simulink model "Quad_UAV_Dynamics_R2024a"  (R2024a)
settings: Solver=VariableStepAuto  StartTime=0.0  StopTime=inf  RelTol=1e-3
PreLoadFcn:
  | InitVars;
values from neighbouring files (symbols this model uses):
  dragCoeffMov = diag([0.1, 0.1, 0.2])    [InitVars.m]
  g = 9.80665    [InitVars.m]
  m_to_mm = 1000    [InitVars.m]
  mass = 1.0    (= 1)    [InitVars.m]
  ms2_to_mg = 1000 / g    (= 101.971621298)    [InitVars.m]
  ms_to_cms = 100    [InitVars.m]
  ref_height = 488.0    (= 488)    [InitVars.m]
  ref_lat = 47.397742    [InitVars.m]
  ref_lon = 8.545594    [InitVars.m]
  rotorDir = [-1; -1; 1; 1]    [InitVars.m]
  rotorPositions = [ armLength*cos(pi/4), -armLength*sin(pi/4), 0 ... (first row only)    [InitVars.m]
  rotorThrustMax = 5.0    (= 5)    [InitVars.m]
  rotorTimeConst = 0.05    [InitVars.m]
  rotorTorqueMax = 0.05    [InitVars.m]
  SampleTime = 0.005    [InitVars.m]    (also in px4HostTarget_TCPIP_Read.m = -1)
  windVel = [0; 0; 0]    [InitVars.m]
undefined symbols (not defined in the file or in its folder): contact, control, fractalcoef, Payload, uav
libraries: uavmavlinklib x5, simulink x2, sharedtransform x2, aerolibatmos2 x1, sensorgpslib x1, robotcorelib x1, mspsensorlib x1, shared6dof x1, uavutilslib x1
(part 1 of 2)
settings Model: LastModifiedBy=LOQ
settings OptimizationCC: BlockReduction=off  BooleanDataType=off
settings DebuggingCC: SaveWithParameterizedLinksMsg=none  UnderspecifiedInitializationDetection=Classic  MergeDetectMultiDrivingBlocksExec=none  SignalResolutionControl=TryResolveAllWithWarning
settings HardwareCC: TargetUnknown=on
settings ModelReferenceCC: PropagateSignalLabelsOutOfModel=off

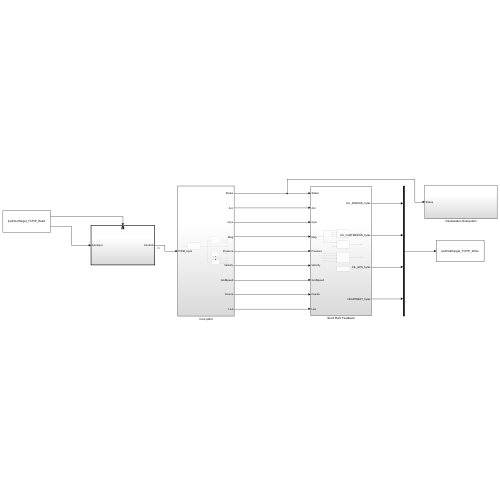
[thumbnail: Simulink's stored preview of the top-level diagram]
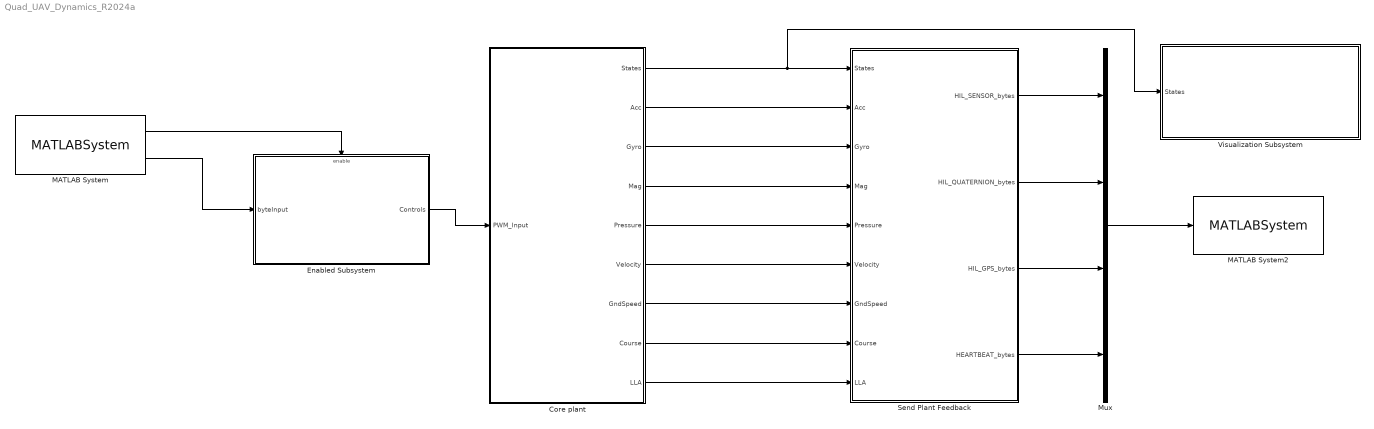
== system Quad_UAV_Dynamics_R2024a ==
  Core plant : Subsystem
  Enabled Subsystem : Subsystem  TreatAsAtomicUnit=on
  MATLAB System : MATLABSystem  System=px4HostTarget_TCPIP_Read  Length=50  SampleTime=SampleTime
      mask Type: px4HostTarget_TCPIP_Read
      mask Display:
      | color('white');
      | plot([100,100,100,100]*1,[100,100,100,100]*1);
      | plot([100,100,100,100]*0,[100,100,100,100]*0);
      | color('black');
      | text(50,50,'TCP Read','horizontalAlignment','center');
      | text(50,12,sprintf('Port: %d',4560) ,'horizontalAlignment', 'center');
      | port_label('output',1,'Status');
      | port_label('output',2,'Data');
  MATLAB System2 : MATLABSystem  System=px4HostTarget_TCPIP_Write
      mask Type: px4HostTarget_TCPIP_Write
      mask Display:
      | color('white');
      | plot([100,100,100,100]*1,[100,100,100,100]*1);
      | plot([100,100,100,100]*0,[100,100,100,100]*0);
      | color('black');
      | sppkgroot = strrep(codertarget.pixhawk.internal.getSpPkgRootDir(),'\','/');
      | image(fullfile(sppkgroot,'resources','TCP.jpg'),'center')
      | color('black');
      | text(50,12,sprintf('Port: %d',4560) ,'horizontalAlignment', 'center');
  Mux : Mux
  Send Plant Feedback : Subsystem
  Visualization Subsystem : Subsystem
  wires:
  MATLAB System/1 -> Enabled Subsystem/Enable
  MATLAB System/2 -> Enabled Subsystem/1(byteInput)
  Enabled Subsystem/1(Controls) -> Core plant/1(PWM_Input)
  Core plant/2(Acc) -> Send Plant Feedback/2(Acc)
  Core plant/3(Gyro) -> Send Plant Feedback/3(Gyro)
  Core plant/4(Mag) -> Send Plant Feedback/4(Mag)
  Core plant/1(States) -> Visualization Subsystem/1(States), Send Plant Feedback/1(States)
  Core plant/5(Pressure) -> Send Plant Feedback/5(Pressure)
  Core plant/6(Velocity) -> Send Plant Feedback/6(Velocity)
  Core plant/7(GndSpeed) -> Send Plant Feedback/7(GndSpeed)
  Core plant/8(Course) -> Send Plant Feedback/8(Course)
  Core plant/9(LLA) -> Send Plant Feedback/9(LLA)
  Send Plant Feedback/1(HIL_SENSOR_bytes) -> Mux/1
  Send Plant Feedback/2(HIL_QUATERNION_bytes) -> Mux/2
  Send Plant Feedback/3(HIL_GPS_bytes) -> Mux/3
  Send Plant Feedback/4(HEARTBEAT_bytes) -> Mux/4
  Mux/1 -> MATLAB System2/1

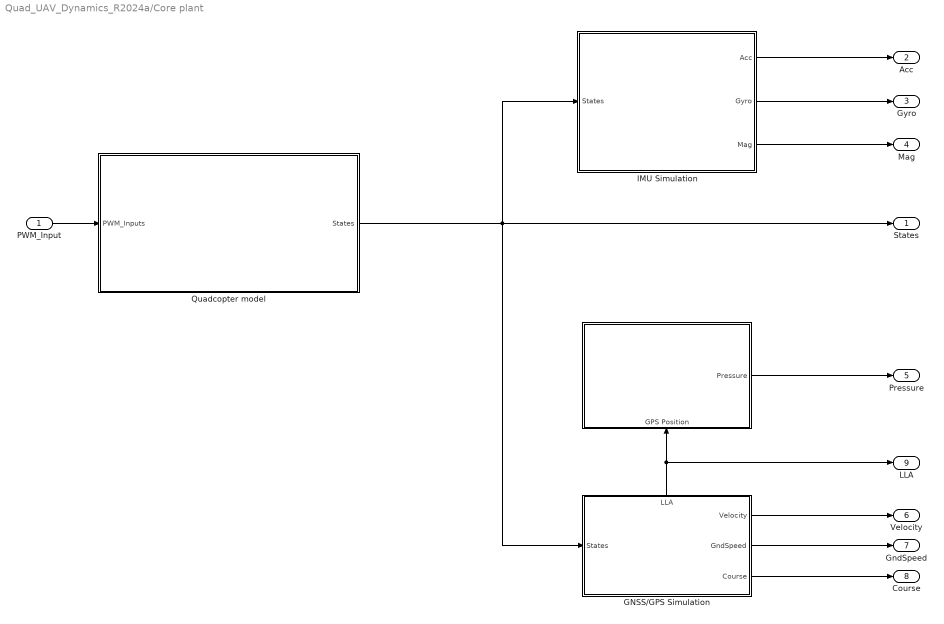
== system Quad_UAV_Dynamics_R2024a/Core plant ==
  PWM_Input : Inport  OutDataTypeStr=double  PortDimensions=[1 4]
  " " : Subsystem
      settings: PortSchema="{\"entries\":[{\"content\":{\"sides\":[{\"content\":{\"connectorIds\":[]},\"type\":\"ConnectorPlacement.EquallySpacedRectSide\",\"uuid\":\"7ecc8b21-8f8f-4144-826a-6b68e30dbf7d\"},{\"content\":{\"connectorIds\":[\"Out1\"],\"side\":\"RIGHT\"},\"type\":\"ConnectorPlacement.EquallySpacedRectSide\",\"uuid\":\"81a1dd55-8330-4386-9921-36c0eb60d526\"},{\"content\":{\"connectorIds\":[],\"side\":\"TOP\"},\"type\":\"ConnectorPlacement.EquallySpacedRectSide\",\"uuid\":\"b99caff5-b40d-407d-b30e-35210c1aee1d\"},{\"content\":{\"connectorIds\":[\"In1\"],\"side\":\"BOTTOM\"},\"type\":\"ConnectorPlacement.EquallySpacedRectSide\",\"uuid\":\"18bfda3d-4fab-4e61-9ebc-e384e51de306\"}]},\"type\":\"ConnectorPlacement.EquallySpacedConnector\",\"uuid\":\"17ab4e96-b761-4c62-a0bb-ab626dac3eaa\"}],\"packageUris\":[\"http://schema.mathworks.com/mf0/Connector/R2020b\"],\"version\":\"1.0\"}"
  GNSS/GPS Simulation : Subsystem
      settings: PortSchema="{\"entries\":[{\"content\":{\"sides\":[{\"content\":{\"connectorIds\":[\"In1\"]},\"type\":\"ConnectorPlacement.EquallySpacedRectSide\",\"uuid\":\"4934e8ff-5d4b-4e11-968d-c23bd62383a0\"},{\"content\":{\"connectorIds\":[\"Out1\",\"Out2\",\"Out3\"],\"side\":\"RIGHT\"},\"type\":\"ConnectorPlacement.EquallySpacedRectSide\",\"uuid\":\"9ec8bc0a-2d3c-4dca-835c-010ac29b6ebc\"},{\"content\":{\"connectorIds\":[\"Out4\"],\"side\":\"TOP\"},\"type\":\"ConnectorPlacement.EquallySpacedRectSide\",\"uuid\":\"04f09eb4-1bd9-450e-b951-47054bdd92ad\"}]},\"type\":\"ConnectorPlacement.EquallySpacedConnector\",\"uuid\":\"9a5920cf-a58d-4c98-839b-fbac94edbe7e\"}],\"packageUris\":[\"http://schema.mathworks.com/mf0/Connector/R2020b\"],\"version\":\"1.0\"}"
  IMU Simulation : Subsystem
      settings: PortSchema="{\"entries\":[{\"content\":{\"sides\":[{\"content\":{},\"type\":\"ConnectorPlacement.EquallySpacedRectSide\",\"uuid\":\"0f5c2282-ad4e-4c27-a92f-532c88dd9b34\"},{\"content\":{\"side\":\"RIGHT\"},\"type\":\"ConnectorPlacement.EquallySpacedRectSide\",\"uuid\":\"b1a389a9-bd19-4f0a-ab56-19663216dbdf\"},{\"content\":{\"connectorIds\":[\"In1\"],\"side\":\"TOP\"},\"type\":\"ConnectorPlacement.EquallySpacedRectSide\",\"uuid\":\"61bb26dd-3b4e-45d7-8996-b1e12f9a0a9d\"},{\"content\":{\"connectorIds\":[\"Out1\",\"Out2\",\"Out3\"],\"side\":\"BOTTOM\"},\"type\":\"ConnectorPlacement.EquallySpacedRectSide\",\"uuid\":\"ba157af1-2ca4-4452-bdd7-6e3dad9cb5e7\"},{\"content\":{\"side\":\"HIDDEN\"},\"type\":\"ConnectorPlacement.EquallySpacedRectSide\",\"uuid\":\"fff182b3-fe96-4082-825e-95746cd3e6b2\"}]},\"type\":\"ConnectorPlacement.EquallySpacedConnector\",\"uuid\":\"8a88afc7-c2a2-4beb-8758-d3390628bed4\"}],\"packageUris\":[\"http://schema.mathworks.com/mf0/Connector/R2020b\"],\"version\":\"1.0\"}"
  Quadcopter model : Subsystem
  States : Outport
  Acc : Outport  Port=2
  Gyro : Outport  Port=3
  Mag : Outport  Port=4
  Pressure : Outport  Port=5
  Velocity : Outport  Port=6
  GndSpeed : Outport  Port=7
  Course : Outport  Port=8
  LLA : Outport  Port=9
  wires:
  IMU Simulation/3(Acc) -> Acc/1
  PWM_Input/1 -> Quadcopter model/1(PWM_Inputs)
  Quadcopter model/1(States) -> GNSS/GPS Simulation/1(States), States/1, IMU Simulation/1(States)
  IMU Simulation/2(Gyro) -> Gyro/1
  IMU Simulation/1(Mag) -> Mag/1
  GNSS/GPS Simulation/4(LLA) -> LLA/1, " "/1(GPS Position)
  " "/1(Pressure) -> Pressure/1
  GNSS/GPS Simulation/1(Velocity) -> Velocity/1
  GNSS/GPS Simulation/2(GndSpeed) -> GndSpeed/1
  GNSS/GPS Simulation/3(Course) -> Course/1

== system Quad_UAV_Dynamics_R2024a/Enabled Subsystem ==
  byteInput : Inport
  Enable : EnablePort
  Bus Selector : BusSelector  OutputSignals=Payload.controls
  Data Type Conversion : DataTypeConversion  OutDataTypeStr=double  SaturateOnIntegerOverflow=off  RndMeth=Floor
  Display : Display
  MAVLink Deserializer : uavmavlinklib/MAVLink Deserializer  dialectSource=Select from standard MAVLink dialects  dialect=common.xml  dialectCustom=common.xml  version=2  messageType=HIL_ACTUATOR_CONTROLS  inputDataLength=off  SystemIDFilter=off  systemID=1  ComponentIDFilter=off  componentID=1  queueMsg=off  queueMsgSize=50  dropNum=off
  Selector1 : Selector  InputPortWidth=16  IndexOptions=Index vector (dialog)  Indices=[1:4]  OutputSizes=1
  Controls : Outport
  wires:
  byteInput/1 -> MAVLink Deserializer/1
  MAVLink Deserializer/2 -> Bus Selector/1
  Bus Selector/1 -> Data Type Conversion/1  "<controls>"
  MAVLink Deserializer/1 -> Display/1  "status"
  Data Type Conversion/1 -> Selector1/1
  Selector1/1 -> Controls/1

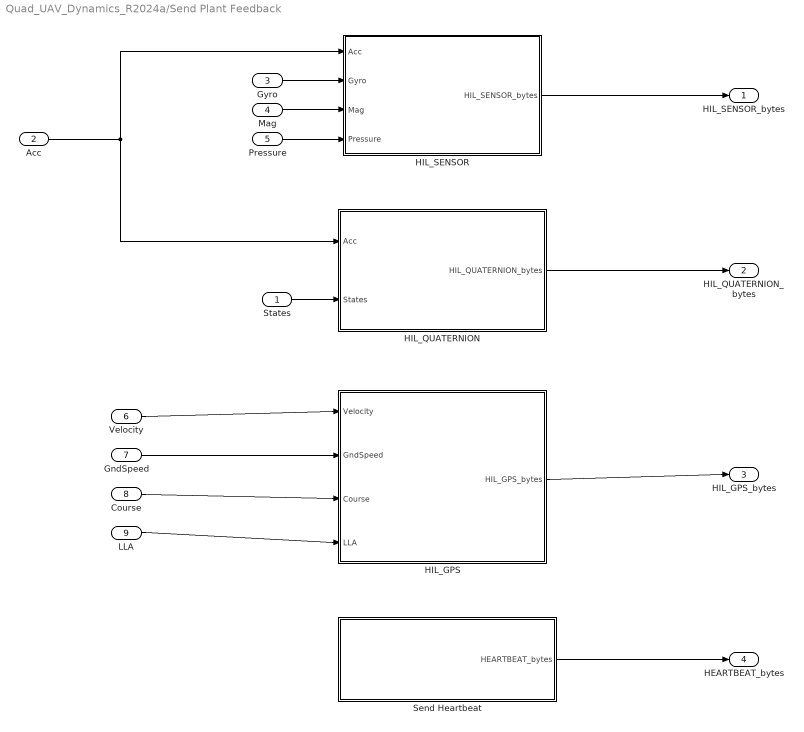
== system Quad_UAV_Dynamics_R2024a/Send Plant Feedback ==
  States : Inport
  Acc : Inport  Port=2
  Gyro : Inport  Port=3
  Mag : Inport  Port=4
  Pressure : Inport  Port=5
  Velocity : Inport  Port=6
  GndSpeed : Inport  Port=7
  Course : Inport  Port=8
  LLA : Inport  Port=9
  HIL_GPS : Subsystem
  HIL_QUATERNION : Subsystem
  HIL_SENSOR : Subsystem
  Send Heartbeat : Subsystem
  HIL_SENSOR_bytes : Outport
  HIL_QUATERNION_bytes : Outport  Port=2
  HIL_GPS_bytes : Outport  Port=3
  HEARTBEAT_bytes : Outport  Port=4
  wires:
  Pressure/1 -> HIL_SENSOR/4(Pressure)
  Acc/1 -> HIL_SENSOR/1(Acc), HIL_QUATERNION/1(Acc)
  States/1 -> HIL_QUATERNION/2(States)
  Mag/1 -> HIL_SENSOR/3(Mag)
  GndSpeed/1 -> HIL_GPS/2(GndSpeed)
  Gyro/1 -> HIL_SENSOR/2(Gyro)
  HIL_SENSOR/1(HIL_SENSOR_bytes) -> HIL_SENSOR_bytes/1
  HIL_QUATERNION/1(HIL_QUATERNION_bytes) -> HIL_QUATERNION_bytes/1
  Course/1 -> HIL_GPS/3(Course)
  Velocity/1 -> HIL_GPS/1(Velocity)
  LLA/1 -> HIL_GPS/4(LLA)
  HIL_GPS/1(HIL_GPS_bytes) -> HIL_GPS_bytes/1
  Send Heartbeat/1(HEARTBEAT_bytes) -> HEARTBEAT_bytes/1

== system Quad_UAV_Dynamics_R2024a/Visualization Subsystem ==
  States : Inport
  Bus Selector : BusSelector  OutputSignals=X,Y,Z  OutputAsBus=on
  Bus Selector1 : BusSelector  OutputSignals=yaw,pitch,roll  OutputAsBus=on
  Rotation Angles to Quaternions : sharedtransform/Rotation Angles to Quaternions  rotationOrder=ZYX  aMode=aMode
  UAV Animation : uavutilslib/UAV Animation  UAVType=Multirotor  UAVSize=1  InertialZDirection=Down  SampleTime=-1
  wires:
  Bus Selector/1 -> UAV Animation/1
  Rotation Angles to Quaternions/1 -> UAV Animation/2
  Bus Selector1/1 -> Rotation Angles to Quaternions/1
  States/1 -> Bus Selector1/1, Bus Selector/1

== system Quad_UAV_Dynamics_R2024a/Core plant/  ==
  GPS Position : Inport
  Extract Altitude : Selector  InputPortWidth=3  IndexOptions=Index vector (dialog)  Indices=[3]  OutputSizes=1
  Gain1 : Gain  Gain=1/m_to_mm
  Gain2 : Gain  Gain=m_to_mm
  Lapse Rate Model : aerolibatmos2/ISA Atmosphere Model  useExtended=off  action=Warning  custom=on  viscosityOut=off  g=9.80665  gamma=1.4  R=287.0531  L=0.0065  h_trop=11000  h_strat=20000  rho0=1.225  P0=101325  T0=288.15  h0=0  S=110.4  Tref=273.15  muref=1.716e-5
  Random Number1 : RandomNumber  Variance=10000  Seed=10  SampleTime=SampleTime
  Sum1 : Sum  Inputs=|++
  Terminator : Terminator
  Terminator1 : Terminator
  Terminator2 : Terminator
  Pressure : Outport
  wires:
  Lapse Rate Model/2 -> Terminator1/1
  Lapse Rate Model/4 -> Terminator2/1
  Lapse Rate Model/1 -> Terminator/1
  Lapse Rate Model/3 -> Pressure/1
  Sum1/1 -> Gain1/1
  Gain2/1 -> Sum1/1
  Extract Altitude/1 -> Gain2/1
  Gain1/1 -> Lapse Rate Model/1
  GPS Position/1 -> Extract Altitude/1
  Random Number1/1 -> Sum1/2  "Pressure_noise"

== system Quad_UAV_Dynamics_R2024a/Core plant/GNSS//GPS Simulation ==
  States : Inport
  Bus Selector : BusSelector  OutputSignals=dx,dy,dz  OutputAsBus=on
  Bus Selector1 : BusSelector  OutputSignals=X,Y,Z  OutputAsBus=on
  GPS : sensorgpslib/GPS  DispRefFrame=NED  PositionInputFormat=Local  ReferenceLocation=[ref_lat ref_lon ref_height]  HorizontalPositionAccuracy=0.01  VerticalPositionAccuracy=0.01  VelocityAccuracy=0.01  DecayFactor=0.99  SeedDouble=67  SimulateUsing=Interpreted execution
  Reshape1 : Reshape  OutputDimensionality=Row vector (2-D)
  Reshape3 : Reshape  OutputDimensionality=Row vector (2-D)
  Velocity : Outport
  GndSpeed : Outport  Port=2
  Course : Outport  Port=3
  LLA : Outport  Port=4
  wires:
  Reshape3/1 -> GPS/1
  GPS/1 -> LLA/1  "lla"
  Bus Selector1/1 -> Reshape3/1
  Bus Selector/1 -> Reshape1/1
  Reshape1/1 -> GPS/2
  GPS/2 -> Velocity/1
  States/1 -> Bus Selector/1, Bus Selector1/1
  GPS/3 -> GndSpeed/1
  GPS/4 -> Course/1

== system Quad_UAV_Dynamics_R2024a/Core plant/IMU Simulation ==
  States : Inport
  IMU Subsystem : Subsystem
  Mag : Outport
  Gyro : Outport  Port=2
  Acc : Outport  Port=3
  wires:
  States/1 -> IMU Subsystem/1(States)
  IMU Subsystem/1(Acc) -> Acc/1
  IMU Subsystem/2(Gyro) -> Gyro/1
  IMU Subsystem/3(Mag) -> Mag/1

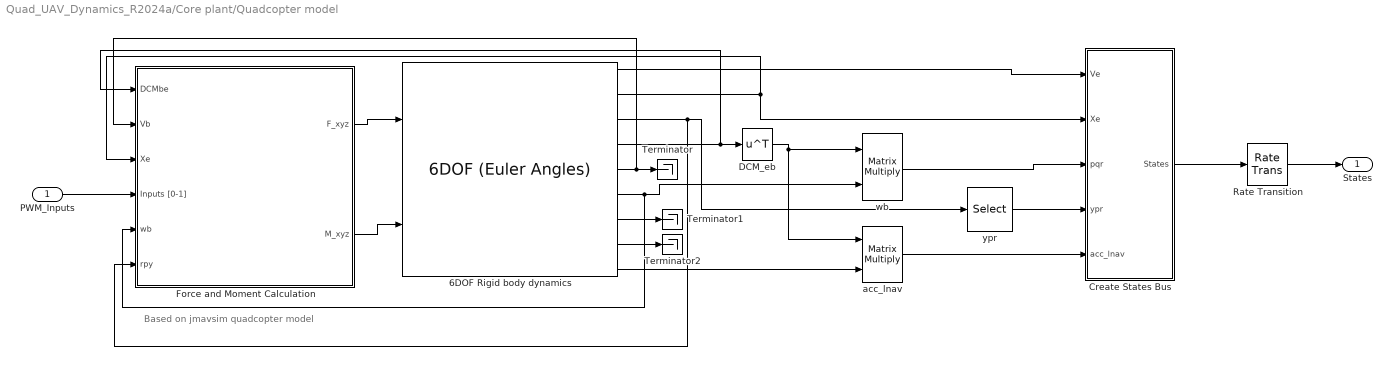
== system Quad_UAV_Dynamics_R2024a/Core plant/Quadcopter model ==
  note: Based on jmavsim quadcopter model
  PWM_Inputs : Inport
  "6DOF Rigid body dynamics " : shared6dof/6DOF (Euler Angles)  units=Metric (MKS)  mtype=Fixed  rep=Euler Angles  xme_0=init.posNED  Vm_0=init.vb  eul_0=init.euler  pm_0=init.angRates  mass_0=mass  mass_e=0.5  mass_f=2.0  inertia=inertia  inertia_e=eye(3)  inertia_f=2*eye(3)  k_quat=Vehicle.SixDOF.quatGain  vre_flag=on  abi_flag=on  aMode=aMode  xme_statename=''  Vm_statename=''  eul_statename=''  quat_statename=''  pm_statename=''  mass_statename=''
  Create States Bus : Subsystem
  DCM_eb : Math  Operator=transpose
  Force and Moment Calculation : Subsystem
  Rate Transition : RateTransition  OutPortSampleTime=SampleTime
  Terminator : Terminator
  Terminator1 : Terminator
  Terminator2 : Terminator
  acc_lnav : Product  Multiplication=Matrix(*)
  wb : Product  Multiplication=Matrix(*)
  ypr : Selector  InputPortWidth=3  IndexOptions=Index vector (dialog)  Indices=[3 2 1]  OutputSizes=1
  States : Outport
  wires:
  "6DOF Rigid body dynamics "/3 -> Force and Moment Calculation/6(rpy), ypr/1
  Force and Moment Calculation/1(F_xyz) -> "6DOF Rigid body dynamics "/1
  Force and Moment Calculation/2(M_xyz) -> "6DOF Rigid body dynamics "/2
  Rate Transition/1 -> States/1
  "6DOF Rigid body dynamics "/1 -> Create States Bus/1(Ve)
  PWM_Inputs/1 -> Force and Moment Calculation/4(Inputs [0-1])
  ypr/1 -> Create States Bus/4(ypr)
  Create States Bus/1(States) -> Rate Transition/1
  "6DOF Rigid body dynamics "/4 -> DCM_eb/1, Force and Moment Calculation/1(DCMbe)
  "6DOF Rigid body dynamics "/2 -> Force and Moment Calculation/3(Xe), Create States Bus/2(Xe)
  "6DOF Rigid body dynamics "/6 -> Force and Moment Calculation/5(wb), wb/2
  wb/1 -> Create States Bus/3(pqr)
  DCM_eb/1 -> acc_lnav/1, wb/1
  "6DOF Rigid body dynamics "/9 -> acc_lnav/2
  acc_lnav/1 -> Create States Bus/5(acc_lnav)
  "6DOF Rigid body dynamics "/5 -> Force and Moment Calculation/2(Vb), Terminator/1
  "6DOF Rigid body dynamics "/7 -> Terminator1/1
  "6DOF Rigid body dynamics "/8 -> Terminator2/1

== system Quad_UAV_Dynamics_R2024a/Send Plant Feedback/HIL_GPS ==
  Velocity : Inport
  GndSpeed : Inport  Port=2
  Course : Inport  Port=3
  LLA : Inport  Port=4
  HIL_GPS Subsystem : Subsystem
  MAVLink Serializer3 : uavmavlinklib/MAVLink Serializer  dialectSource=Select from standard MAVLink dialects  dialect=common.xml  dialectCustom=common.xml  version=2  messageType=HIL_GPS
  Terminator3 : Terminator
  HIL_GPS_bytes : Outport
  wires:
  Course/1 -> HIL_GPS Subsystem/4(Course)
  Velocity/1 -> HIL_GPS Subsystem/2(Velocity)
  MAVLink Serializer3/2 -> Terminator3/1
  HIL_GPS Subsystem/1(Out1) -> MAVLink Serializer3/1
  MAVLink Serializer3/1 -> HIL_GPS_bytes/1
  LLA/1 -> HIL_GPS Subsystem/1(LLA)
  GndSpeed/1 -> HIL_GPS Subsystem/3(GndSpeed)

== system Quad_UAV_Dynamics_R2024a/Send Plant Feedback/HIL_QUATERNION ==
  Acc : Inport
  States : Inport  Port=2
  GPS Subsystem : Subsystem
      settings: PortSchema="{\"entries\":[{\"content\":{\"sides\":[{\"content\":{\"connectorIds\":[\"In1\"]},\"type\":\"ConnectorPlacement.EquallySpacedRectSide\",\"uuid\":\"bd7d303d-974a-4dd9-8d27-04cf87176bd7\"},{\"content\":{\"connectorIds\":[\"Out1\"],\"side\":\"RIGHT\"},\"type\":\"ConnectorPlacement.EquallySpacedRectSide\",\"uuid\":\"9b60b4cf-af27-4ca7-86b7-e75d27668f15\"},{\"content\":{\"connectorIds\":[\"In2\"],\"side\":\"TOP\"},\"type\":\"ConnectorPlacement.EquallySpacedRectSide\",\"uuid\":\"cd4d20a6-3033-4c65-942d-f02a7fa933e8\"},{\"content\":{\"side\":\"BOTTOM\"},\"type\":\"ConnectorPlacement.EquallySpacedRectSide\",\"uuid\":\"d837ff15-3ee7-4ba9-aab0-0378a7633b3a\"},{\"content\":{\"side\":\"HIDDEN\"},\"type\":\"ConnectorPlacement.EquallySpacedRectSide\",\"uuid\":\"eefe2c49-f98f-4c11-8e75-b071b558b610\"}]},\"type\":\"ConnectorPlacement.EquallySpacedConnector\",\"uuid\":\"bd9fca06-cb18-49af-bec9-4d4823ab7b04\"}],\"packageUris\":[\"http://schema.mathworks.com/mf0/Connector/R2020b\"],\"version\":\"1.0\"}"
  MAVLink Serializer2 : uavmavlinklib/MAVLink Serializer  dialectSource=Select from standard MAVLink dialects  dialect=common.xml  dialectCustom=common.xml  version=2  messageType=HIL_STATE_QUATERNION
  Terminator2 : Terminator
  HIL_QUATERNION_bytes : Outport
  wires:
  States/1 -> GPS Subsystem/1(States)
  MAVLink Serializer2/2 -> Terminator2/1
  GPS Subsystem/1(HIL Quaternion) -> MAVLink Serializer2/1
  MAVLink Serializer2/1 -> HIL_QUATERNION_bytes/1
  Acc/1 -> GPS Subsystem/2(Acc)

== system Quad_UAV_Dynamics_R2024a/Send Plant Feedback/HIL_SENSOR ==
  Acc : Inport
  Gyro : Inport  Port=2
  Mag : Inport  Port=3
  Pressure : Inport  Port=4
  Hil Sensor Creation subsystem : Subsystem
  MAVLink Serializer1 : uavmavlinklib/MAVLink Serializer  dialectSource=Select from standard MAVLink dialects  dialect=common.xml  dialectCustom=common.xml  version=2  messageType=HIL_SENSOR
  Terminator1 : Terminator
  HIL_SENSOR_bytes : Outport
  wires:
  MAVLink Serializer1/2 -> Terminator1/1
  Hil Sensor Creation subsystem/1(HIL Sensor) -> MAVLink Serializer1/1
  Acc/1 -> Hil Sensor Creation subsystem/1(Acc)
  MAVLink Serializer1/1 -> HIL_SENSOR_bytes/1
  Gyro/1 -> Hil Sensor Creation subsystem/2(Gyro)
  Mag/1 -> Hil Sensor Creation subsystem/3(Mag)
  Pressure/1 -> Hil Sensor Creation subsystem/4(Pressure)

== system Quad_UAV_Dynamics_R2024a/Send Plant Feedback/Send Heartbeat ==
  Bus Assignment : BusAssignment  AssignedSignals=Payload.autopilot,Payload.type
  Constant : Constant  SampleTime=SampleTime
  Constant1 : Constant  Value=12  SampleTime=SampleTime
  Data Type Conversion : DataTypeConversion  OutDataTypeStr=uint8  SaturateOnIntegerOverflow=off  RndMeth=Floor
  Data Type Conversion1 : DataTypeConversion  OutDataTypeStr=uint8  SaturateOnIntegerOverflow=off  RndMeth=Floor
  MAVLink Blank Message : Subsystem  InitFcn=uav.sluav.internal.mavlink.util.errorIfBlocksConflict(bdroot(gcb))  mask(MAVLink Blank Message){dialectSource=Select from standard MAVLink dialects, dialect=common.xml, dialectCustom=common.xml, version=2, messageType=HEARTBEAT, SystemID=2, ComponentID=51, SampleTime=SampleTime}
      mask prompts: dialectSource "uav:robotsluav:mavlink:DialectSourcePrompt"; dialect "uav:robotsluav:mavlink:DialectPrompt"; dialectCustom "uav:robotsluav:mavlink:DialectPromptCustom"; version "uav:robotsluav:mavlink:VersionPrompt"; messageType "uav:robotsluav:mavlink:MessageTypePrompt"; SystemID "uav:robotsluav:mavlink:EnterSystemIDPrompt"; ComponentID "uav:robotsluav:mavlink:EnterComponentIDPrompt"; SampleTime "Simulink:blkprm_prompts:AllSrcBlksSampleTime"
      mask help: uav:robotsluav:mavlink:BlankMessageDescription
      mask init:
      | uav.sluav.internal.mavlink.block.MessageBlockMask.dispatch('maskInitialize', gcb)
      settings: LibrarySourceBlock=uavmavlinklib/MAVLink Blank Message  ModelCloseFcn=uav.sluav.internal.mavlink.block.MessageBlockMask.dispatch('modelCloseFcn', gcb);
      mask Help: eval("helpview('uav','uavMAVLinkBlankMessage')");
      mask TypeOptions dialectSource: uav:robotsluav:mavlink:DialectSourceFromStandard | uav:robotsluav:mavlink:DialectSourceSpecifyOwn
      mask Callback dialectSource: uav.sluav.internal.mavlink.block.MessageBlockMask.dispatch('dialectSourceSelect', gcb);
      mask TypeOptions dialect: uav:robotsluav:mavlink:DialectCommon | uav:robotsluav:mavlink:DialectArdupilotmega | uav:robotsluav:mavlink:DialectASLUAV | uav:robotsluav:mavlink:DialectAutoquad | uav:robotsluav:mavlink:DialectIcarous | uav:robotsluav:mavlink:DialectMatrixpilot | uav:robotsluav:mavlink:DialectMinimal | uav:robotsluav:mavlink:DialectPaparazzi | uav:robotsluav:mavlink:DialectSlugs | uav:robotsluav:mavlink:DialectStandard | uav:robotsluav:mavlink:DialectUalberta | uav:robotsluav:mavlink:DialectUAvionix
      mask Callback dialect: uav.sluav.internal.mavlink.block.MessageBlockMask.dispatch('dialectEdit', gcb);
      mask Callback dialectCustom: uav.sluav.internal.mavlink.block.MessageBlockMask.dispatch('dialectEdit', gcb);
      mask TypeOptions version: 2 | 1
      mask Callback version: uav.sluav.internal.mavlink.block.MessageBlockMask.dispatch('versionEdit', gcb);
      mask Callback messageType: uav.sluav.internal.mavlink.block.MessageBlockMask.dispatch('messageTypeEdit', gcb);
      mask Callback SystemID: uav.sluav.internal.mavlink.block.MessageBlockMask.dispatch('updateSystemAndComponentID', gcb);
      mask Callback ComponentID: uav.sluav.internal.mavlink.block.MessageBlockMask.dispatch('updateSystemAndComponentID', gcb);
      mask TypeOptions SampleTime: MsgIDConstant/SampleTime
      mask DialogControl MainContainer Prompt: uav:robotsluav:mavlink:MainTabTitle
      mask DialogControl dialectSource Prompt: MAVLink dialect source:
      mask DialogControl dialect Prompt: MAVLink dialect:
      mask DialogControl dialectCustom Prompt: MAVLink dialect:
      mask DialogControl dialectBrowseButton Prompt: uav:robotsluav:mavlink:DialectBrowsePrompt
      mask DialogControl dialectBrowseButton Callback: uav.sluav.internal.mavlink.block.MessageBlockMask.dispatch('dialectBrowse', gcb);
      mask DialogControl version Prompt: MAVLink version:
      mask DialogControl messageType Prompt: MAVLink message type:
      mask DialogControl msgSelectButton Prompt: uav:robotsluav:mavlink:MessageSelectPrompt
      mask DialogControl msgSelectButton Callback: uav.sluav.internal.mavlink.block.MessageBlockMask.dispatch('messageTypeSelect', gcb, 'uav.sluav.internal.mavlink.dlg.MessageTypeSelector');
      mask DialogControl SystemID Prompt: System ID:
      mask DialogControl ComponentID Prompt: Component ID:
      mask DialogControl SampleTime Prompt: Sample time:
      mask Display:
      | color('black');
      | text(0.5, 0.10, 'HEARTBEAT', 'horizontalAlignment', 'center');
      | port_label('output', 1, 'Msg');
  MAVLink Serializer : uavmavlinklib/MAVLink Serializer  dialectSource=Select from standard MAVLink dialects  dialect=common.xml  dialectCustom=common.xml  version=2  messageType=HEARTBEAT
  Terminator4 : Terminator
  HEARTBEAT_bytes : Outport
  wires:
  Bus Assignment/1 -> MAVLink Serializer/1
  Constant/1 -> Data Type Conversion/1
  MAVLink Serializer/1 -> HEARTBEAT_bytes/1
  Data Type Conversion1/1 -> Bus Assignment/3
  Data Type Conversion/1 -> Bus Assignment/2
  MAVLink Serializer/2 -> Terminator4/1
  Constant1/1 -> Data Type Conversion1/1
  MAVLink Blank Message/1(Out1) -> Bus Assignment/1

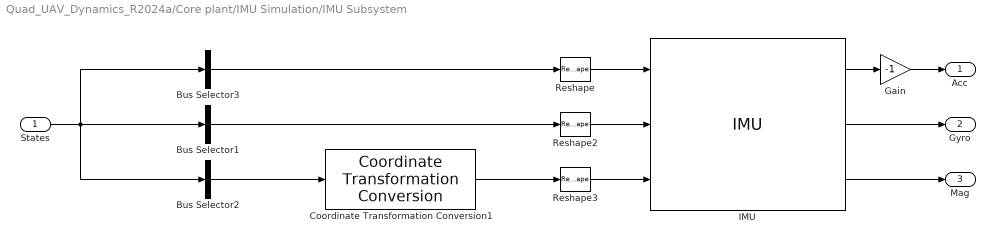
== system Quad_UAV_Dynamics_R2024a/Core plant/IMU Simulation/IMU Subsystem ==
  States : Inport
  Bus Selector1 : BusSelector  OutputSignals=p,q,r  OutputAsBus=on
  Bus Selector2 : BusSelector  OutputSignals=yaw,pitch,roll  OutputAsBus=on
  Bus Selector3 : BusSelector  OutputSignals=ddx,ddy,ddz  OutputAsBus=on
  Coordinate Transformation Conversion1 : robotcorelib/Coordinate Transformation Conversion  InputRepresentation=Euler Angles  InputEulerSequence=ZYX  ShowTrVecInputPort=on  OutputRepresentation=Quaternion  OutputEulerSequence=ZYX  ShowTrVecOutputPort=on  SimulateUsing=Interpreted execution
  Gain : Gain  Gain=-1
  IMU : mspsensorlib/IMU  DispRefFrame=NED  TemperaturePort=off  Temperature=25  MagneticFieldPort=off  MagneticFieldNED=[ 27.5550, -2.4169, -16.0849 ]  MagneticFieldENU=[ -2.4169, 27.5550, 16.0849 ]  SeedDouble=67  SimulateUsing=Interpreted execution  AccelParamsMeasurementRange=Inf  AccelParamsResolution=0  AccelParamsConstantBias=[ 0, 0, 0 ]  AccelParamsAxesMisalignment=[ 0, 0, 0 ]  AccelParamsNoiseDensity=[ 0, 0, 0 ]  AccelParamsBiasInstability=[ 0, 0, 0 ]  AccelParamsBiasInstabilityNumerator=fractalcoef().Numerator  AccelParamsBiasInstabilityDenominator=fractalcoef().Denominator  AccelParamsRandomWalk=[ 0, 0, 0 ]  AccelParamsNoiseType=double-sided  AccelParamsTemperatureBias=[ 0, 0, 0 ]  AccelParamsTemperatureScaleFactor=[ 0, 0, 0 ]  GyroParamsMeasurementRange=Inf  GyroParamsResolution=0  GyroParamsConstantBias=[ 0, 0, 0 ]  GyroParamsAxesMisalignment=[ 0, 0, 0 ]  GyroParamsAccelerationBias=[ 0, 0, 0 ]  GyroParamsNoiseDensity=[ 0, 0, 0 ]  GyroParamsBiasInstability=[ 0, 0, 0 ]  GyroParamsBiasInstabilityNumerator=fractalcoef().Numerator  GyroParamsBiasInstabilityDenominator=fractalcoef().Denominator  GyroParamsRandomWalk=[ 0, 0, 0 ]  GyroParamsNoiseType=double-sided  GyroParamsTemperatureBias=[ 0, 0, 0 ]  GyroParamsTemperatureScaleFactor=[ 0, 0, 0 ]  MagParamsMeasurementRange=Inf  MagParamsResolution=0  MagParamsConstantBias=[ 0, 0, 0 ]  MagParamsAxesMisalignment=[ 0, 0, 0 ]  MagParamsNoiseDensity=[ 0, 0, 0 ]  MagParamsBiasInstability=[ 0, 0, 0 ]  MagParamsBiasInstabilityNumerator=fractalcoef().Numerator  MagParamsBiasInstabilityDenominator=fractalcoef().Denominator  MagParamsRandomWalk=[ 0, 0, 0 ]  MagParamsNoiseType=double-sided  MagParamsTemperatureBias=[ 0, 0, 0 ]  MagParamsTemperatureScaleFactor=[ 0, 0, 0 ]
  Reshape : Reshape  OutputDimensionality=Row vector (2-D)
  Reshape2 : Reshape  OutputDimensionality=Row vector (2-D)
  Reshape3 : Reshape  OutputDimensionality=Row vector (2-D)
  Acc : Outport
  Gyro : Outport  Port=2
  Mag : Outport  Port=3
  wires:
  Bus Selector1/1 -> Reshape2/1
  IMU/1 -> Gain/1
  Bus Selector2/1 -> Coordinate Transformation Conversion1/1
  IMU/3 -> Mag/1
  Reshape2/1 -> IMU/2
  Bus Selector3/1 -> Reshape/1
  Coordinate Transformation Conversion1/1 -> Reshape3/1
  Reshape/1 -> IMU/1
  IMU/2 -> Gyro/1
  Reshape3/1 -> IMU/3
  States/1 -> Bus Selector3/1, Bus Selector2/1, Bus Selector1/1
  Gain/1 -> Acc/1

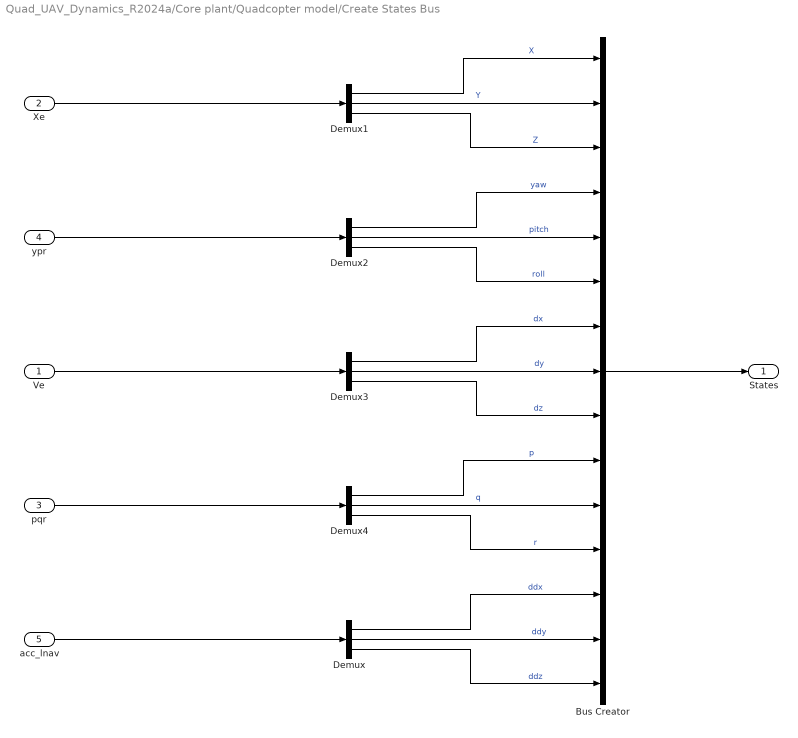
== system Quad_UAV_Dynamics_R2024a/Core plant/Quadcopter model/Create States Bus ==
  Ve : Inport
  Xe : Inport  Port=2
  pqr : Inport  Port=3
  ypr : Inport  Port=4
  acc_lnav : Inport  Port=5
  Bus Creator : BusCreator  Inputs=15
  Demux{,1..4} (5 alike) : Demux  Outputs=3
  States : Outport
  wires:
  Demux1/1 -> Bus Creator/1  "X"
  Demux1/2 -> Bus Creator/2  "Y"
  ypr/1 -> Demux2/1
  Demux2/2 -> Bus Creator/5  "pitch"
  Demux3/2 -> Bus Creator/8  "dy"
  Demux2/3 -> Bus Creator/6  "roll"
  pqr/1 -> Demux4/1
  Ve/1 -> Demux3/1
  Demux2/1 -> Bus Creator/4  "yaw"
  Demux1/3 -> Bus Creator/3  "Z"
  Demux3/1 -> Bus Creator/7  "dx"
  Demux4/2 -> Bus Creator/11  "q"
  Demux3/3 -> Bus Creator/9  "dz"
  Demux4/3 -> Bus Creator/12  "r"
  Demux4/1 -> Bus Creator/10  "p"
  Bus Creator/1 -> States/1
  Xe/1 -> Demux1/1
  acc_lnav/1 -> Demux/1
  Demux/3 -> Bus Creator/15  "ddz"
  Demux/2 -> Bus Creator/14  "ddy"
  Demux/1 -> Bus Creator/13  "ddx"

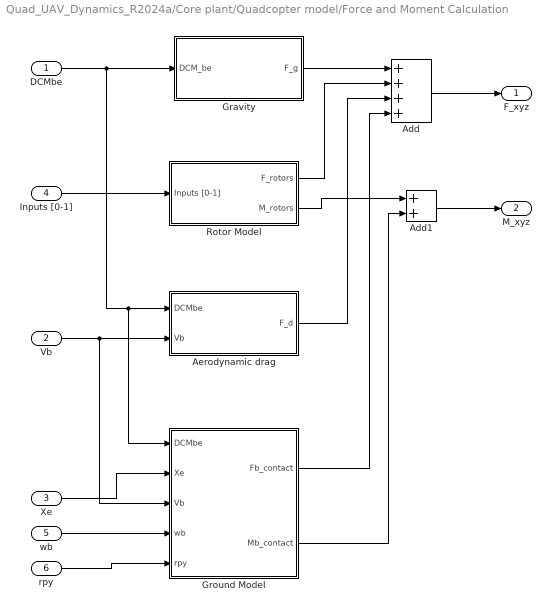
== system Quad_UAV_Dynamics_R2024a/Core plant/Quadcopter model/Force and Moment Calculation ==
  DCMbe : Inport
  Vb : Inport  Port=2
  Xe : Inport  Port=3
  Inputs [0-1] : Inport  Port=4
  wb : Inport  Port=5
  rpy : Inport  Port=6
  Add : Sum  Inputs=++++
  Add1 : Sum
  Aerodynamic drag : Subsystem
  Gravity : Subsystem
  Ground Model : Subsystem
  Rotor Model : Subsystem
  F_xyz : Outport
  M_xyz : Outport  Port=2
  wires:
  Inputs [0-1]/1 -> Rotor Model/1(Inputs [0-1])
  Gravity/1(F_g) -> Add/1
  Add/1 -> F_xyz/1
  Rotor Model/1(F_rotors) -> Add/2
  Aerodynamic drag/1(F_d) -> Add/3
  Ground Model/1(Fb_contact) -> Add/4
  Vb/1 -> Ground Model/3(Vb), Aerodynamic drag/2(Vb)
  DCMbe/1 -> Ground Model/1(DCMbe), Aerodynamic drag/1(DCMbe), Gravity/1(DCM_be)
  Xe/1 -> Ground Model/2(Xe)
  wb/1 -> Ground Model/4(wb)
  rpy/1 -> Ground Model/5(rpy)
  Rotor Model/2(M_rotors) -> Add1/1
  Ground Model/2(Mb_contact) -> Add1/2
  Add1/1 -> M_xyz/1

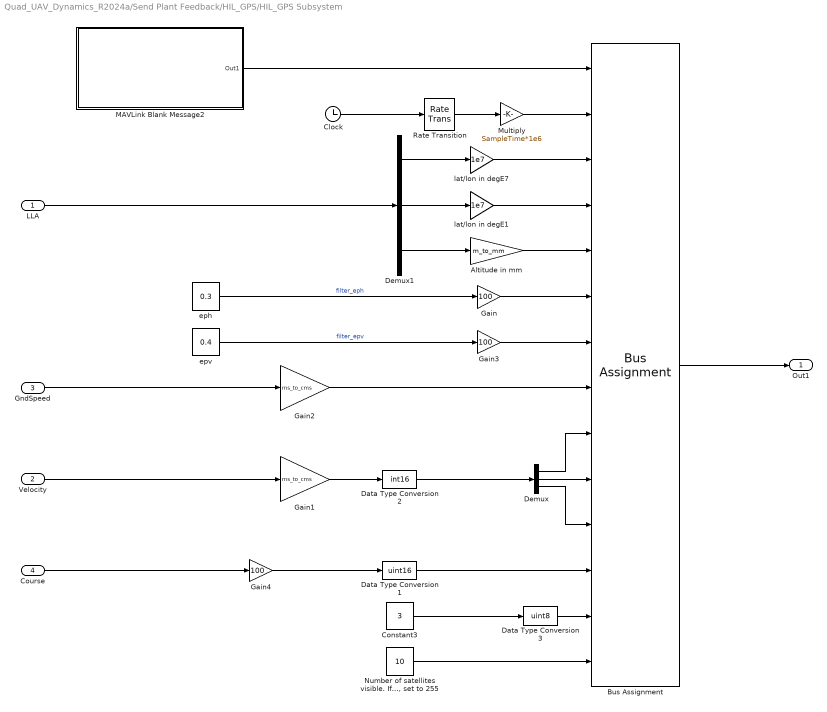
== system Quad_UAV_Dynamics_R2024a/Send Plant Feedback/HIL_GPS/HIL_GPS Subsystem ==
  LLA : Inport
  Velocity : Inport  Port=2
  GndSpeed : Inport  Port=3
  Course : Inport  Port=4
  Altitude in mm : Gain  Gain=m_to_mm  OutDataTypeStr=Inherit: Inherit via back propagation
  Bus Assignment : BusAssignment  AssignedSignals=Payload.time_usec,Payload.lat,Payload.lon,Payload.alt,Payload.eph,Payload.epv,Payload.vel,Payload.vn,Payload.ve,Payload.vd,Payload.cog,Payload.fix_type,Payload.satellites_visible
  Clock : Clock
  Constant3 : Constant  Value=3  OutDataTypeStr=Inherit: Inherit via back propagation  SampleTime=-1
  Data Type Conversion1 : DataTypeConversion  OutDataTypeStr=uint16  SaturateOnIntegerOverflow=off  RndMeth=Floor
  Data Type Conversion2 : DataTypeConversion  OutDataTypeStr=int16  SaturateOnIntegerOverflow=off  RndMeth=Floor
  Data Type Conversion3 : DataTypeConversion  OutDataTypeStr=uint8  SaturateOnIntegerOverflow=off  RndMeth=Floor
  Demux : Demux  Outputs=3
  Demux1 : Demux  Outputs=3
  Gain : Gain  Gain=100  OutDataTypeStr=Inherit: Inherit via back propagation
  Gain1 : Gain  Gain=ms_to_cms
  Gain2 : Gain  Gain=ms_to_cms  OutDataTypeStr=uint16
  Gain3 : Gain  Gain=100  OutDataTypeStr=Inherit: Inherit via back propagation
  Gain4 : Gain  Gain=100
  MAVLink Blank Message2 : Subsystem  InitFcn=uav.sluav.internal.mavlink.util.errorIfBlocksConflict(bdroot(gcb))  mask(MAVLink Blank Message){dialectSource=Select from standard MAVLink dialects, dialect=common.xml, dialectCustom=common.xml, version=2, messageType=HIL_GPS, SystemID=2, ComponentID=51, SampleTime=SampleTime}
      mask prompts: dialectSource "uav:robotsluav:mavlink:DialectSourcePrompt"; dialect "uav:robotsluav:mavlink:DialectPrompt"; dialectCustom "uav:robotsluav:mavlink:DialectPromptCustom"; version "uav:robotsluav:mavlink:VersionPrompt"; messageType "uav:robotsluav:mavlink:MessageTypePrompt"; SystemID "uav:robotsluav:mavlink:EnterSystemIDPrompt"; ComponentID "uav:robotsluav:mavlink:EnterComponentIDPrompt"; SampleTime "Simulink:blkprm_prompts:AllSrcBlksSampleTime"
      mask help: uav:robotsluav:mavlink:BlankMessageDescription
      mask init:
      | uav.sluav.internal.mavlink.block.MessageBlockMask.dispatch('maskInitialize', gcb)
      settings: LibrarySourceBlock=uavmavlinklib/MAVLink Blank Message  ModelCloseFcn=uav.sluav.internal.mavlink.block.MessageBlockMask.dispatch('modelCloseFcn', gcb);
      mask Help: eval("helpview('uav','uavMAVLinkBlankMessage')");
      mask TypeOptions dialectSource: uav:robotsluav:mavlink:DialectSourceFromStandard | uav:robotsluav:mavlink:DialectSourceSpecifyOwn
      mask Callback dialectSource: uav.sluav.internal.mavlink.block.MessageBlockMask.dispatch('dialectSourceSelect', gcb);
      mask TypeOptions dialect: uav:robotsluav:mavlink:DialectCommon | uav:robotsluav:mavlink:DialectArdupilotmega | uav:robotsluav:mavlink:DialectASLUAV | uav:robotsluav:mavlink:DialectAutoquad | uav:robotsluav:mavlink:DialectIcarous | uav:robotsluav:mavlink:DialectMatrixpilot | uav:robotsluav:mavlink:DialectMinimal | uav:robotsluav:mavlink:DialectPaparazzi | uav:robotsluav:mavlink:DialectSlugs | uav:robotsluav:mavlink:DialectStandard | uav:robotsluav:mavlink:DialectUalberta | uav:robotsluav:mavlink:DialectUAvionix
      mask Callback dialect: uav.sluav.internal.mavlink.block.MessageBlockMask.dispatch('dialectEdit', gcb);
      mask Callback dialectCustom: uav.sluav.internal.mavlink.block.MessageBlockMask.dispatch('dialectEdit', gcb);
      mask TypeOptions version: 2 | 1
      mask Callback version: uav.sluav.internal.mavlink.block.MessageBlockMask.dispatch('versionEdit', gcb);
      mask Callback messageType: uav.sluav.internal.mavlink.block.MessageBlockMask.dispatch('messageTypeEdit', gcb);
      mask Callback SystemID: uav.sluav.internal.mavlink.block.MessageBlockMask.dispatch('updateSystemAndComponentID', gcb);
      mask Callback ComponentID: uav.sluav.internal.mavlink.block.MessageBlockMask.dispatch('updateSystemAndComponentID', gcb);
      mask TypeOptions SampleTime: MsgIDConstant/SampleTime
      mask DialogControl MainContainer Prompt: uav:robotsluav:mavlink:MainTabTitle
      mask DialogControl dialectSource Prompt: MAVLink dialect source:
      mask DialogControl dialect Prompt: MAVLink dialect:
      mask DialogControl dialectCustom Prompt: MAVLink dialect:
      mask DialogControl dialectBrowseButton Prompt: uav:robotsluav:mavlink:DialectBrowsePrompt
      mask DialogControl dialectBrowseButton Callback: uav.sluav.internal.mavlink.block.MessageBlockMask.dispatch('dialectBrowse', gcb);
      mask DialogControl version Prompt: MAVLink version:
      mask DialogControl messageType Prompt: MAVLink message type:
      mask DialogControl msgSelectButton Prompt: uav:robotsluav:mavlink:MessageSelectPrompt
      mask DialogControl msgSelectButton Callback: uav.sluav.internal.mavlink.block.MessageBlockMask.dispatch('messageTypeSelect', gcb, 'uav.sluav.internal.mavlink.dlg.MessageTypeSelector');
      mask DialogControl SystemID Prompt: System ID:
      mask DialogControl ComponentID Prompt: Component ID:
      mask DialogControl SampleTime Prompt: Sample time:
      mask Display:
      | color('black');
      | text(0.5, 0.10, 'HIL_GPS', 'horizontalAlignment', 'center');
      | port_label('output', 1, 'Msg');
  Multiply : Gain  Gain=SampleTime*1e6  OutDataTypeStr=Inherit: Inherit via back propagation
  "Number of satellites visible. If unknown, set to 255" : Constant  Value=10  OutDataTypeStr=Inherit: Inherit via back propagation  SampleTime=-1
  Rate Transition : RateTransition
  eph : Constant  Value=0.3  SampleTime=-1
  epv : Constant  Value=0.4  SampleTime=-1
  lat/lon in degE1 : Gain  Gain=1e7  OutDataTypeStr=Inherit: Inherit via back propagation
  lat/lon in degE7 : Gain  Gain=1e7  OutDataTypeStr=Inherit: Inherit via back propagation
  Out1 : Outport
  wires:
  Gain2/1 -> Bus Assignment/8
  lat/lon in degE7/1 -> Bus Assignment/3
  Demux1/1 -> lat/lon in degE7/1
  Demux/3 -> Bus Assignment/11
  MAVLink Blank Message2/1(Out1) -> Bus Assignment/1
  Gain1/1 -> Data Type Conversion2/1
  Demux1/3 -> Altitude in mm/1
  Demux1/2 -> lat/lon in degE1/1
  Demux/1 -> Bus Assignment/9
  lat/lon in degE1/1 -> Bus Assignment/4
  Altitude in mm/1 -> Bus Assignment/5
  Data Type Conversion2/1 -> Demux/1
  Demux/2 -> Bus Assignment/10
  Bus Assignment/1 -> Out1/1
  "Number of satellites visible. If unknown, set to 255"/1 -> Bus Assignment/14
  Gain/1 -> Bus Assignment/6
  Gain3/1 -> Bus Assignment/7
  LLA/1 -> Demux1/1
  GndSpeed/1 -> Gain2/1
  Velocity/1 -> Gain1/1
  Course/1 -> Gain4/1
  Data Type Conversion1/1 -> Bus Assignment/12
  eph/1 -> Gain/1  "filter_eph"
  epv/1 -> Gain3/1  "filter_epv"
  Data Type Conversion3/1 -> Bus Assignment/13
  Gain4/1 -> Data Type Conversion1/1
  Constant3/1 -> Data Type Conversion3/1
  Clock/1 -> Rate Transition/1
  Rate Transition/1 -> Multiply/1
  Multiply/1 -> Bus Assignment/2

== system Quad_UAV_Dynamics_R2024a/Send Plant Feedback/HIL_QUATERNION/GPS Subsystem ==
  States : Inport
  Acc : Inport  Port=2
  HIL Quaternion Creation Subsystem : Subsystem
  HIL Quaternion : Outport
  wires:
  HIL Quaternion Creation Subsystem/1(HIL Quaternion) -> HIL Quaternion/1
  States/1 -> HIL Quaternion Creation Subsystem/2(States)
  Acc/1 -> HIL Quaternion Creation Subsystem/1(Acc)

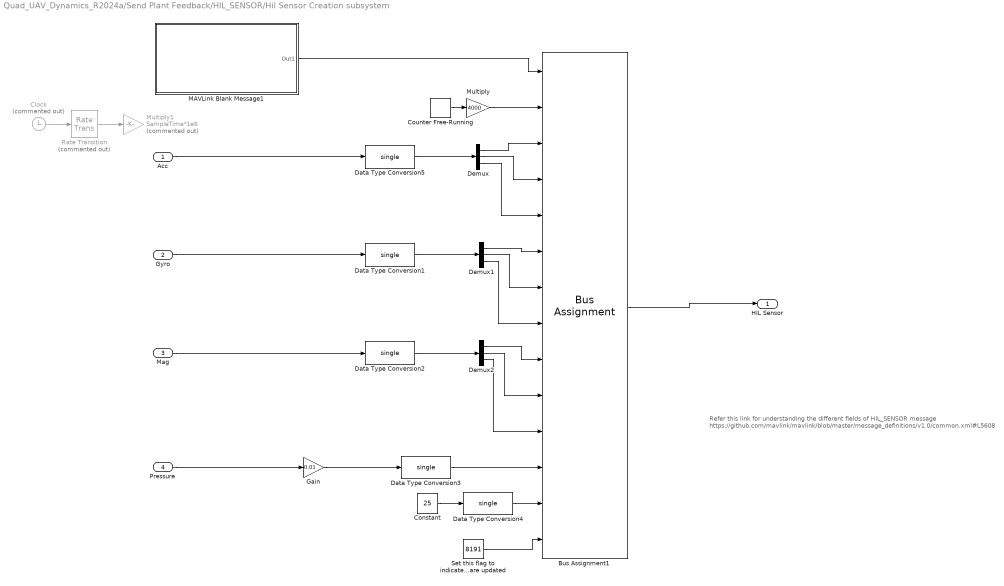
== system Quad_UAV_Dynamics_R2024a/Send Plant Feedback/HIL_SENSOR/Hil Sensor Creation subsystem ==
  note: Refer this link for understanding the different fields of HIL_SENSOR message https://github.com/mavlink/mavlink/blob/master/message_definitions/v1.0/common.xml#L5608
  Acc : Inport
  Gyro : Inport  Port=2
  Mag : Inport  Port=3
  Pressure : Inport  Port=4
  Bus Assignment1 : BusAssignment  AssignedSignals=Payload.time_usec,Payload.xacc,Payload.yacc,Payload.zacc,Payload.xgyro,Payload.ygyro,Payload.zgyro,Payload.xmag,Payload.ymag,Payload.zmag,Payload.abs_pressure,Payload.temperature,Payload.fields_updated
  Clock : Clock  Commented=on
  Constant : Constant  Value=25
  Counter Free-Running : simulink/Sources/Counter Free-Running  NumBits=64  tsamp=SampleTime
  Data Type Conversion{1..5} (5 alike) : DataTypeConversion  OutDataTypeStr=single  SaturateOnIntegerOverflow=off  RndMeth=Floor
  Demux : Demux  Outputs=3
  Demux1 : Demux  Outputs=3
  Demux2 : Demux  Outputs=3
  Gain : Gain  Gain=0.01
  MAVLink Blank Message1 : Subsystem  InitFcn=uav.sluav.internal.mavlink.util.errorIfBlocksConflict(bdroot(gcb))  mask(MAVLink Blank Message){dialectSource=Select from standard MAVLink dialects, dialect=common.xml, dialectCustom=common.xml, version=2, messageType=HIL_SENSOR, SystemID=2, ComponentID=51, SampleTime=SampleTime}
      mask prompts: dialectSource "uav:robotsluav:mavlink:DialectSourcePrompt"; dialect "uav:robotsluav:mavlink:DialectPrompt"; dialectCustom "uav:robotsluav:mavlink:DialectPromptCustom"; version "uav:robotsluav:mavlink:VersionPrompt"; messageType "uav:robotsluav:mavlink:MessageTypePrompt"; SystemID "uav:robotsluav:mavlink:EnterSystemIDPrompt"; ComponentID "uav:robotsluav:mavlink:EnterComponentIDPrompt"; SampleTime "Simulink:blkprm_prompts:AllSrcBlksSampleTime"
      mask help: uav:robotsluav:mavlink:BlankMessageDescription
      mask init:
      | uav.sluav.internal.mavlink.block.MessageBlockMask.dispatch('maskInitialize', gcb)
      settings: LibrarySourceBlock=uavmavlinklib/MAVLink Blank Message  ModelCloseFcn=uav.sluav.internal.mavlink.block.MessageBlockMask.dispatch('modelCloseFcn', gcb);
      mask Help: eval("helpview('uav','uavMAVLinkBlankMessage')");
      mask TypeOptions dialectSource: uav:robotsluav:mavlink:DialectSourceFromStandard | uav:robotsluav:mavlink:DialectSourceSpecifyOwn
      mask Callback dialectSource: uav.sluav.internal.mavlink.block.MessageBlockMask.dispatch('dialectSourceSelect', gcb);
      mask TypeOptions dialect: uav:robotsluav:mavlink:DialectCommon | uav:robotsluav:mavlink:DialectArdupilotmega | uav:robotsluav:mavlink:DialectASLUAV | uav:robotsluav:mavlink:DialectAutoquad | uav:robotsluav:mavlink:DialectIcarous | uav:robotsluav:mavlink:DialectMatrixpilot | uav:robotsluav:mavlink:DialectMinimal | uav:robotsluav:mavlink:DialectPaparazzi | uav:robotsluav:mavlink:DialectSlugs | uav:robotsluav:mavlink:DialectStandard | uav:robotsluav:mavlink:DialectUalberta | uav:robotsluav:mavlink:DialectUAvionix
      mask Callback dialect: uav.sluav.internal.mavlink.block.MessageBlockMask.dispatch('dialectEdit', gcb);
      mask Callback dialectCustom: uav.sluav.internal.mavlink.block.MessageBlockMask.dispatch('dialectEdit', gcb);
      mask TypeOptions version: 2 | 1
      mask Callback version: uav.sluav.internal.mavlink.block.MessageBlockMask.dispatch('versionEdit', gcb);
      mask Callback messageType: uav.sluav.internal.mavlink.block.MessageBlockMask.dispatch('messageTypeEdit', gcb);
      mask Callback SystemID: uav.sluav.internal.mavlink.block.MessageBlockMask.dispatch('updateSystemAndComponentID', gcb);
      mask Callback ComponentID: uav.sluav.internal.mavlink.block.MessageBlockMask.dispatch('updateSystemAndComponentID', gcb);
      mask TypeOptions SampleTime: MsgIDConstant/SampleTime
      mask DialogControl MainContainer Prompt: uav:robotsluav:mavlink:MainTabTitle
      mask DialogControl dialectSource Prompt: MAVLink dialect source:
      mask DialogControl dialect Prompt: MAVLink dialect:
      mask DialogControl dialectCustom Prompt: MAVLink dialect:
      mask DialogControl dialectBrowseButton Prompt: uav:robotsluav:mavlink:DialectBrowsePrompt
      mask DialogControl dialectBrowseButton Callback: uav.sluav.internal.mavlink.block.MessageBlockMask.dispatch('dialectBrowse', gcb);
      mask DialogControl version Prompt: MAVLink version:
      mask DialogControl messageType Prompt: MAVLink message type:
      mask DialogControl msgSelectButton Prompt: uav:robotsluav:mavlink:MessageSelectPrompt
      mask DialogControl msgSelectButton Callback: uav.sluav.internal.mavlink.block.MessageBlockMask.dispatch('messageTypeSelect', gcb, 'uav.sluav.internal.mavlink.dlg.MessageTypeSelector');
      mask DialogControl SystemID Prompt: System ID:
      mask DialogControl ComponentID Prompt: Component ID:
      mask DialogControl SampleTime Prompt: Sample time:
      mask Display:
      | color('black');
      | text(0.5, 0.10, 'HIL_SENSOR', 'horizontalAlignment', 'center');
      | port_label('output', 1, 'Msg');
  Multiply : Gain  Gain=4000  OutDataTypeStr=Inherit: Inherit via back propagation
  Multiply1 : Gain  Commented=on  Gain=SampleTime*1e6  OutDataTypeStr=Inherit: Inherit via back propagation
  Rate Transition : RateTransition  Commented=on
  Set this flag to indicate all flags are updated : Constant  Value=8191  OutDataTypeStr=Inherit: Inherit via back propagation  SampleTime=SampleTime
  HIL Sensor : Outport
  wires:
  Data Type Conversion2/1 -> Demux2/1
  Demux1/1 -> Bus Assignment1/6
  Counter Free-Running/1 -> Multiply/1
  Demux1/3 -> Bus Assignment1/8
  Data Type Conversion1/1 -> Demux1/1
  Gyro/1 -> Data Type Conversion1/1
  Bus Assignment1/1 -> HIL Sensor/1
  Set this flag to indicate all flags are updated/1 -> Bus Assignment1/14
  Demux/3 -> Bus Assignment1/5
  Demux2/2 -> Bus Assignment1/10
  Demux2/3 -> Bus Assignment1/11
  Data Type Conversion5/1 -> Demux/1
  Demux/1 -> Bus Assignment1/3
  MAVLink Blank Message1/1(Out1) -> Bus Assignment1/1
  Demux2/1 -> Bus Assignment1/9
  Demux/2 -> Bus Assignment1/4
  Demux1/2 -> Bus Assignment1/7
  Acc/1 -> Data Type Conversion5/1
  Mag/1 -> Data Type Conversion2/1
  Data Type Conversion3/1 -> Bus Assignment1/12
  Gain/1 -> Data Type Conversion3/1
  Pressure/1 -> Gain/1
  Constant/1 -> Data Type Conversion4/1
  Data Type Conversion4/1 -> Bus Assignment1/13
  Rate Transition/1 -> Multiply1/1
  Clock/1 -> Rate Transition/1
  Multiply/1 -> Bus Assignment1/2

== system Quad_UAV_Dynamics_R2024a/Send Plant Feedback/Send Heartbeat/MAVLink Blank Message ==
  ComponentIDConstant : Constant  Value=51  OutDataTypeStr=uint8  SampleTime=-1
  MAVLinkMsgBusCreator : BusCreator  Inputs=5  OutDataTypeStr=Bus: SL_Bus_MAVLink_HEARTBEAT_Packet  NonVirtualBus=on
  MsgIDConstant : Constant  Value=0  OutDataTypeStr=uint32  SampleTime=SampleTime
  MsgModifier : MATLABSystem  System=uav.sluav.internal.system.MAVLinkMsgModifier  SLBusName=SL_Bus_MAVLink_HEARTBEAT_Payload
      mask Type: uav.sluav.internal.system.MAVLinkMsgModifier
      mask Display:
      | disp('MAVLinkMsgModifier');
      | port_label('input',1,'msgID');
      | port_label('input',2,'inputBusStruct');
      | port_label('output',1,'modifiedBusStruct');
  PayloadConstant : Constant  Value=0  OutDataTypeStr=Bus: SL_Bus_MAVLink_HEARTBEAT_Payload  SampleTime=-1
  SequenceConstant : Constant  Value=0  OutDataTypeStr=uint8  SampleTime=-1
  SystemIDConstant : Constant  Value=2  OutDataTypeStr=uint8  SampleTime=-1
  Out1 : Outport
  wires:
  MsgModifier/1 -> MAVLinkMsgBusCreator/5  "Payload"
  MAVLinkMsgBusCreator/1 -> Out1/1
  MsgIDConstant/1 -> MsgModifier/1, MAVLinkMsgBusCreator/1  "MsgID"
  SystemIDConstant/1 -> MAVLinkMsgBusCreator/2  "SystemID"
  ComponentIDConstant/1 -> MAVLinkMsgBusCreator/3  "ComponentID"
  SequenceConstant/1 -> MAVLinkMsgBusCreator/4  "Sequence"
  PayloadConstant/1 -> MsgModifier/2  "Payload"

== system Quad_UAV_Dynamics_R2024a/Core plant/Quadcopter model/Force and Moment Calculation/Aerodynamic drag ==
  DCMbe : Inport
  Vb : Inport  Port=2
  Constant : Constant  Value=windVel
  Constant1 : Constant  Value=dragCoeffMov
  calcDragVector : MATLAB Function  TreatAsAtomicUnit=on
  gain : Gain  Gain=-1
  relative air velocity (body frame) : Sum
  wind (body frame) : Product  Multiplication=Matrix(*)
  F_d : Outport
  wires:
  Vb/1 -> gain/1
  calcDragVector/1(dragVec) -> F_d/1
  relative air velocity (body frame)/1 -> calcDragVector/1(airVel)
  gain/1 -> relative air velocity (body frame)/2
  Constant1/1 -> calcDragVector/2(dragCoeff)
  DCMbe/1 -> wind (body frame)/1
  Constant/1 -> wind (body frame)/2
  wind (body frame)/1 -> relative air velocity (body frame)/1

== system Quad_UAV_Dynamics_R2024a/Core plant/Quadcopter model/Force and Moment Calculation/Gravity ==
  DCM_be : Inport
  Constant : Constant  Value=[0 0 g]'
  Gain : Gain  Gain=mass
  Matrix Multiply : Product  Multiplication=Matrix(*)
  F_g : Outport
  wires:
  Matrix Multiply/1 -> Gain/1
  Constant/1 -> Matrix Multiply/2
  DCM_be/1 -> Matrix Multiply/1
  Gain/1 -> F_g/1

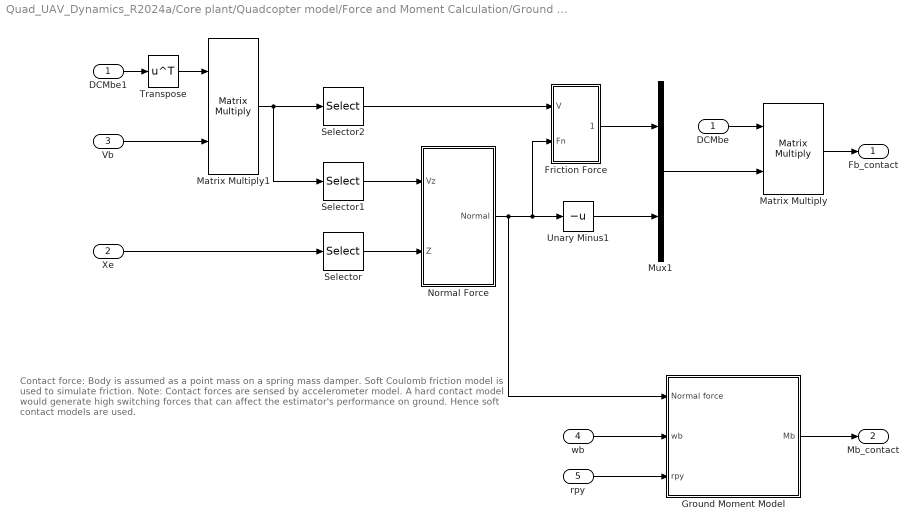
== system Quad_UAV_Dynamics_R2024a/Core plant/Quadcopter model/Force and Moment Calculation/Ground Model ==
  note: Contact force:
      | Body is assumed as a point mass on a spring mass damper. Soft Coulomb friction model is used to simulate friction.
      |
      | Note:
      | Contact forces are sensed by accelerometer model. A hard contact model would generate high switching forces that can affect the estimator's performance on ground. Hence soft contact models are used.
  DCMbe : Inport
  Xe : Inport  Port=2
  Vb : Inport  Port=3
  wb : Inport  Port=4
  rpy : Inport  Port=5
  DCMbe1 : InportShadow
  Friction Force : Subsystem
  Ground Moment Model : Subsystem
  Matrix Multiply : Product  Multiplication=Matrix(*)
  Matrix Multiply1 : Product  Multiplication=Matrix(*)
  Mux1 : Mux  Inputs=2
  Normal Force : Subsystem
  Selector : Selector  InputPortWidth=3  IndexOptions=Index vector (dialog)  Indices=[3]  OutputSizes=1
  Selector1 : Selector  InputPortWidth=3  IndexOptions=Index vector (dialog)  Indices=[3]  OutputSizes=1
  Selector2 : Selector  InputPortWidth=3  IndexOptions=Index vector (dialog)  Indices=[1,2]  OutputSizes=1
  Transpose : Math  Operator=transpose
  Unary Minus1 : UnaryMinus
  Fb_contact : Outport
  Mb_contact : Outport  Port=2
  wires:
  Xe/1 -> Selector/1
  Selector1/1 -> Normal Force/1(Vz)
  Selector/1 -> Normal Force/2(Z)
  DCMbe/1 -> Matrix Multiply/1
  Matrix Multiply/1 -> Fb_contact/1
  Normal Force/1(Normal) -> Ground Moment Model/1(Normal force), Unary Minus1/1, Friction Force/2(Fn)
  Mux1/1 -> Matrix Multiply/2
  Unary Minus1/1 -> Mux1/2
  Selector2/1 -> Friction Force/1(V)
  Friction Force/1(Friction) -> Mux1/1
  DCMbe1/1 -> Transpose/1
  Transpose/1 -> Matrix Multiply1/1
  Vb/1 -> Matrix Multiply1/2
  Matrix Multiply1/1 -> Selector1/1, Selector2/1
  Ground Moment Model/1(Mb) -> Mb_contact/1
  wb/1 -> Ground Moment Model/2(wb)
  rpy/1 -> Ground Moment Model/3(rpy)

== system Quad_UAV_Dynamics_R2024a/Core plant/Quadcopter model/Force and Moment Calculation/Rotor Model ==
  Inputs [0-1] : Inport
  Constant : Constant  Value=rotorPositions
  Constant1 : Constant  Value=rotorDir
  MATLAB Function : MATLAB Function  TreatAsAtomicUnit=on
  Thrust model : Subsystem
  Torque model : Subsystem
  F_rotors : Outport
  M_rotors : Outport  Port=2
  wires:
  Inputs [0-1]/1 -> Torque model/1(In1), Thrust model/1(In1)
  MATLAB Function/1(netF) -> F_rotors/1
  MATLAB Function/2(netM) -> M_rotors/1
  Constant/1 -> MATLAB Function/3(rotorPositions)
  Constant1/1 -> MATLAB Function/4(rotorDir)
  Torque model/1(Out1) -> MATLAB Function/2(tauEachRotor)
  Thrust model/1(Out1) -> MATLAB Function/1(thrustEachRotor)

== system Quad_UAV_Dynamics_R2024a/Send Plant Feedback/HIL_GPS/HIL_GPS Subsystem/MAVLink Blank Message2 ==
  ComponentIDConstant : Constant  Value=51  OutDataTypeStr=uint8  SampleTime=-1
  MAVLinkMsgBusCreator : BusCreator  Inputs=5  OutDataTypeStr=Bus: SL_Bus_MAVLink_HIL_GPS_Packet  NonVirtualBus=on
  MsgIDConstant : Constant  Value=113  OutDataTypeStr=uint32  SampleTime=SampleTime
  MsgModifier : MATLABSystem  System=uav.sluav.internal.system.MAVLinkMsgModifier  SLBusName=SL_Bus_MAVLink_HIL_GPS_Payload
      mask Type: uav.sluav.internal.system.MAVLinkMsgModifier
      mask Display:
      | disp('MAVLinkMsgModifier');
      | port_label('input',1,'msgID');
      | port_label('input',2,'inputBusStruct');
      | port_label('output',1,'modifiedBusStruct');
  PayloadConstant : Constant  Value=0  OutDataTypeStr=Bus: SL_Bus_MAVLink_HIL_GPS_Payload  SampleTime=-1
  SequenceConstant : Constant  Value=0  OutDataTypeStr=uint8  SampleTime=-1
  SystemIDConstant : Constant  Value=2  OutDataTypeStr=uint8  SampleTime=-1
  Out1 : Outport
  wires:
  MsgModifier/1 -> MAVLinkMsgBusCreator/5  "Payload"
  MAVLinkMsgBusCreator/1 -> Out1/1
  MsgIDConstant/1 -> MsgModifier/1, MAVLinkMsgBusCreator/1  "MsgID"
  SystemIDConstant/1 -> MAVLinkMsgBusCreator/2  "SystemID"
  ComponentIDConstant/1 -> MAVLinkMsgBusCreator/3  "ComponentID"
  SequenceConstant/1 -> MAVLinkMsgBusCreator/4  "Sequence"
  PayloadConstant/1 -> MsgModifier/2  "Payload"
